simulink model "H6"  (R2025a)
settings: Solver=VariableStepAuto  StartTime=0.0  StopTime=2  RelTol=1e-3
libraries: spsIGBTDiodeLib x6, spsSeriesRLCBranchLib x4, spsCurrentMeasurementLib x1, spsDCVoltageSourceLib x1, simulink x1, spsVoltageMeasurementLib x1, sps_lib x1
settings Model: Creator=Mohamed Ibrahim  LastModifiedBy=Mohamed Ibrahim

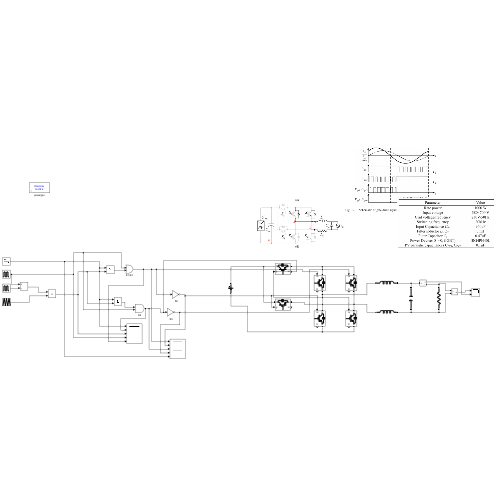
[thumbnail: Simulink's stored preview of the top-level diagram]
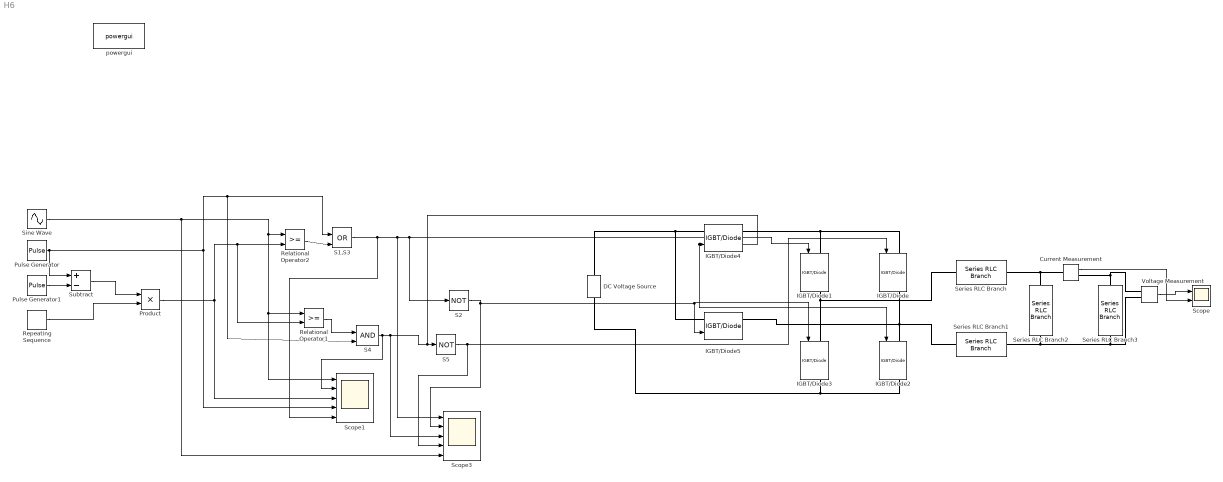
== system H6 ==
  Current Measurement : spsCurrentMeasurementLib/Current Measurement  PhasorSimulation=off  OutputType=Complex  PSBequivalent=0
  DC Voltage Source : spsDCVoltageSourceLib/DC Voltage Source  Amplitude=700  Measurements=None
  IGBT/Diode{,1..5} (6 alike) : spsIGBTDiodeLib/IGBT//Diode  Ron=1e-3  Rs=1e5  Cs=inf  Measurements=on
  Product : Product
  Pulse Generator : DiscretePulseGenerator  PulseType=Time based  Period=0.02  PulseWidth=50
  Pulse Generator1 : DiscretePulseGenerator  PulseType=Time based  Period=0.02  PulseWidth=50  PhaseDelay=0.01
  Relational Operator1 : RelationalOperator  OutDataTypeStr=boolean  RndMeth=Simplest  InputSameDT=off
  Relational Operator2 : RelationalOperator  OutDataTypeStr=boolean  RndMeth=Simplest  InputSameDT=off
  Repeating Sequence : simulink/Sources/Repeating Sequence  rep_seq_t=[0 0.000025 0.00005]  rep_seq_y=[0 1 0]
  S1,S3 : Logic  Operator=OR  IconShape=distinctive  AllPortsSameDT=off  OutDataTypeStr=boolean
  S2 : Logic  Operator=NOT  IconShape=distinctive  AllPortsSameDT=off  OutDataTypeStr=boolean
  S4 : Logic  IconShape=distinctive  AllPortsSameDT=off  OutDataTypeStr=boolean
  S5 : Logic  Operator=NOT  IconShape=distinctive  AllPortsSameDT=off  OutDataTypeStr=boolean
  Scope : Scope  NumInputPorts=2
      settings: ActiveDisplayYMinimum=-418.96250227447428  ActiveDisplayYMaximum=491.62589282071008
  Scope1 : Scope  NumInputPorts=5
      settings: ActiveDisplayString=4  ActiveDisplayYMinimum=-0.12499999999999997  ActiveDisplayYMaximum=1.125
  Scope3 : Scope  NumInputPorts=5
      settings: ActiveDisplayString=4  ActiveDisplayYMinimum=-0.12499999999999997  ActiveDisplayYMaximum=1.125  DataLoggingVariableName=ScopeData3
  Series RLC Branch : spsSeriesRLCBranchLib/Series RLC Branch  LConnTagsString=__new0  RConnTagsString=__new0  BranchType=L  Resistance=1  Inductance=3e-3  SetiL0=off  InitialCurrent=0  Capacitance=1e-6  Setx0=off  InitialVoltage=0  Measurements=None
  Series RLC Branch1 : spsSeriesRLCBranchLib/Series RLC Branch  LConnTagsString=__new0  RConnTagsString=__new0  BranchType=L  Resistance=1  Inductance=3e-3  SetiL0=off  InitialCurrent=0  Capacitance=1e-6  Setx0=off  InitialVoltage=0  Measurements=None
  Series RLC Branch2 : spsSeriesRLCBranchLib/Series RLC Branch  LConnTagsString=__new0  RConnTagsString=__new0  BranchType=C  Resistance=1  Inductance=1e-3  SetiL0=off  InitialCurrent=0  Capacitance=0.47e-6  Setx0=off  InitialVoltage=0  Measurements=None
  Series RLC Branch3 : spsSeriesRLCBranchLib/Series RLC Branch  LConnTagsString=__new0  RConnTagsString=__new0  BranchType=R  Resistance=1  Inductance=1e-3  SetiL0=off  InitialCurrent=0  Capacitance=1e-6  Setx0=off  InitialVoltage=0  Measurements=None
  Sine Wave : Sin  Frequency=100*pi  SampleTime=0
  Subtract : Sum  Inputs=+-
  Voltage Measurement : spsVoltageMeasurementLib/Voltage Measurement  PhasorSimulation=off  OutputType=Complex  PSBequivalent=0
  powergui : sps_lib/powergui  Priority=1  SimulationMode=Discrete  SampleTime=1e-6  frequency=60  Iterations=50  frequencyindice=0  Pbase=100e6  ErrMax=1e-4  UnitsV=kV  UnitsW=MW  buscounter=0  FunctionMessages=off  echomessages=off  EnableUseOfTLC=off  CurrentSourceSwitches=off  DisableSnubberDevices=off  DisableRonSwitches=off  DisableVfSwitches=off  DisplayEquations=off  AutomaticDiscreteSolvers=off  SolverType=Tustin/Backward Euler (TBE)  Interpol=off  ExternalGateDelay=off  methode=off  Ts=100  x0status=blocks  SPID=on  SwTol=0  HookPort=off  NonlinearTolerance=1e-4  nMaxIteration=100  ContinueOnMaxIteration=off  RestoreLinks=warning  ResistiveCurrentMeasurement=off  Frange=[0:2:500]  Ylog=off  Xlog=on  ShowGrid=off  save=off  variable=ZData  structure=0  ZoomFFT=off  StartTime=0.0  cycles=1  DisplayStyle=1  fundamental=60  FreqAxis=off  MaxFrequency=1000  frequencyindicesteady=1  RmsSteady=1  display=off
  wires:
  Voltage Measurement/1 -> Scope/1
  Current Measurement/1 -> Scope/2
  S2/1 -> IGBT/Diode5/1, IGBT/Diode3/1, Scope3/2
  Pulse Generator/1 -> Subtract/1, S4/2, S1,S3/1, Scope1/4
  Relational Operator2/1 -> S1,S3/2
  Product/1 -> Scope1/3, Relational Operator1/2, Relational Operator2/2
  Pulse Generator1/1 -> Subtract/2
  Sine Wave/1 -> Scope3/5, Relational Operator1/1, Scope1/1, Relational Operator2/1
  Relational Operator1/1 -> S4/1
  S5/1 -> IGBT/Diode/1, Scope3/4
  Repeating Sequence/1 -> Product/2
  S1,S3/1 -> IGBT/Diode1/1, S2/1, Scope3/1, Scope1/5
  Subtract/1 -> Product/1
  S4/1 -> Scope1/2, Scope3/3, IGBT/Diode4/1, IGBT/Diode2/1, S5/1
  connections:
  IGBT/Diode5/LConn1 -- IGBT/Diode4/LConn1 -- DC Voltage Source/RConn1
  Series RLC Branch/RConn1 -- Current Measurement/LConn1 -- Series RLC Branch2/LConn1
  Voltage Measurement/LConn2 -- Series RLC Branch3/RConn1 -- Series RLC Branch1/LConn1 -- Series RLC Branch2/RConn1
  IGBT/Diode3/LConn1 -- IGBT/Diode1/RConn1 -- Series RLC Branch/LConn1
  IGBT/Diode2/LConn1 -- IGBT/Diode5/RConn1 -- IGBT/Diode/RConn1 -- Series RLC Branch1/RConn1
  IGBT/Diode2/RConn1 -- DC Voltage Source/LConn1 -- IGBT/Diode3/RConn1
  IGBT/Diode4/RConn1 -- IGBT/Diode1/LConn1 -- IGBT/Diode/LConn1
  Series RLC Branch3/LConn1 -- Voltage Measurement/LConn1 -- Current Measurement/RConn1
